simulink model "Papersimcurrentsource3"  (R2025a)
settings: Solver=ode23tb  StartTime=0.0  StopTime=0.3  MaxStep=5e-5  RelTol=1e-3
undefined symbols (not defined in the file): D11, Delta, I_PV_R_ML
libraries: spsRMSLib x20, spsCurrentMeasurementLib x5, spsParallelRLCLoadLib x4, spsACCurrentSourceLib x3, spsBreakerLib x3, spsPower3phInstantaneousLib x3, spsThreePhaseVIMeasurementLib x3, spsSequenceAnalyzerLib x2, simulink x1, spsMeanLib x1, spsPowerPhasorLib x1, eePowerMeasurement x1
settings Model: NumberOfSteps=2  Creator=ADMIN  LastModifiedBy=Ayush

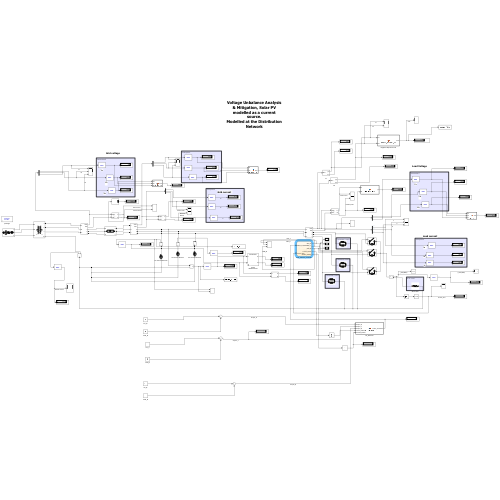
[thumbnail: Simulink's stored preview of the top-level diagram]
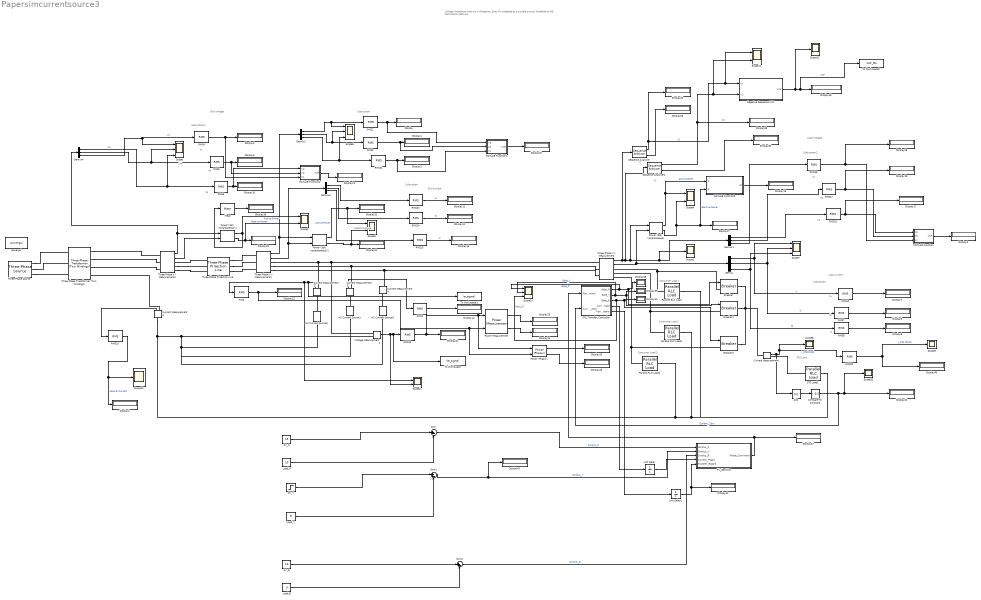
== system Papersimcurrentsource3 ==
  note: Gate_B
  note: Consumer Load 3
  note: Consumer Load 2
  note: STS Load
  note: Consumer Load 1
  note: Reactive Power
  note: V1
  note: Subsystem1
  note: Subsystem2
  note: Voltage Unbalance Analysis & Mitigation, Solar PV modelled as a current source.
      | Modelled at the Distribution Network
  note: Subsystem
  note: Subsystem
  note: Subsystem
  note: Ia
  note: Ib
  note: Ic
  note: Grid voltage
  note: Load current
  note: Load Voltage
  note: Vc
  note: Vb
  note: Va
  note: Vc
  note: Vb
  note: Va
  note: Grid current
  note: V2
  AC Current Source1 : spsACCurrentSourceLib/AC Current Source  Amplitude=20.86  Phase=-150  Frequency=50  SampleTime=0  Measurements=None
      settings: LibrarySourceBlock=sps_lib/Sources/AC Current Source
  AC Current Source2 : spsACCurrentSourceLib/AC Current Source  Amplitude=I_PV_R_ML  Phase=-30  Frequency=50  SampleTime=0  Measurements=None
      settings: LibrarySourceBlock=sps_lib/Sources/AC Current Source
  AC Current Source3 : spsACCurrentSourceLib/AC Current Source  Amplitude=40.86  Phase=90  Frequency=50  SampleTime=0  Measurements=None
      settings: LibrarySourceBlock=sps_lib/Sources/AC Current Source
  Abs : Abs  SaturateOnIntegerOverflow=off
  Breaker : spsBreakerLib/Breaker  InitialState=0  SwitchingTimes="[1/60  5/60]"  External=on  BreakerResistance=0.01  SnubberResistance=1e6  SnubberCapacitance=inf  Measurements=None  MoreParameters=on  NoBreakLoop=off
  Breaker1 : spsBreakerLib/Breaker  InitialState=0  SwitchingTimes="[1/60  5/60]"  External=on  BreakerResistance=0.01  SnubberResistance=1e6  SnubberCapacitance=inf  Measurements=None  MoreParameters=on  NoBreakLoop=off
  Breaker2 : spsBreakerLib/Breaker  InitialState=0  SwitchingTimes="[1/60  5/60]"  External=on  BreakerResistance=0.01  SnubberResistance=1e6  SnubberCapacitance=inf  Measurements=None  MoreParameters=on  NoBreakLoop=off
  Compare To Constant : simulink/Logic and Bit Operations/Compare To Constant  relop=<  const=0.5  OutDataTypeStr=boolean
  Current Measurement{,1..4} (5 alike) : spsCurrentMeasurementLib/Current Measurement  PhasorSimulation=off  OutputType=Complex  PSBequivalent=0
  Demux{,1..4} (5 alike) : Demux  Outputs=3
  Display{,1..27,29..40,42..46} (45 alike) : Display
  Load_B : Constant  Value=3
  Load_R : Constant  Value=10
  Load_Y : Constant  Value=5
  MATLAB Function : MATLAB Function  TreatAsAtomicUnit=on
  MATLAB Function1 : MATLAB Function  TreatAsAtomicUnit=on
  MATLAB Function2 : MATLAB Function  TreatAsAtomicUnit=on
  MATLAB Function3 : MATLAB Function  TreatAsAtomicUnit=on
  Mean : spsMeanLib/Mean  Freq=50  Vinit=0  Ts=0
  Negative-Sequence VUF : MATLAB Function  TreatAsAtomicUnit=on
  PV_B : Constant  Value=10
  PV_Decision : MATLAB Function  TreatAsAtomicUnit=on
  PV_R : Constant  Value=15
  PV_Y : Step  Time=0.1  After=10  SampleTime=0
  Parallel RLC Load : spsParallelRLCLoadLib/Parallel RLC Load  LConnTagsString=a  RConnTagsString=__new0  NominalVoltage=239.6  NominalFrequency=50  ActivePower=P_R_ML  InductivePower=0.0315e3  CapacitivePower=0  Setx0=off  InitialVoltage=0  SetiL0=off  InitialCurrent=0  Measurements=None  LoadType=constant PQ
      settings: AttributesFormatString=\n  LibrarySourceBlock=sps_lib/Passives/Parallel RLC Load
  Parallel RLC Load1 : spsParallelRLCLoadLib/Parallel RLC Load  LConnTagsString=a  RConnTagsString=__new0  NominalVoltage=239.6  NominalFrequency=50  ActivePower=P_Y_ML  InductivePower=0.1700e3  CapacitivePower=0  Setx0=off  InitialVoltage=0  SetiL0=off  InitialCurrent=0  Measurements=None  LoadType=constant PQ
      settings: AttributesFormatString=\n  LibrarySourceBlock=sps_lib/Passives/Parallel RLC Load
  Parallel RLC Load2 : spsParallelRLCLoadLib/Parallel RLC Load  LConnTagsString=a  RConnTagsString=__new0  NominalVoltage=239.6  NominalFrequency=50  ActivePower=P_B_ML  InductivePower=0.0416e3  CapacitivePower=0  Setx0=off  InitialVoltage=0  SetiL0=off  InitialCurrent=0  Measurements=None  LoadType=constant PQ
      settings: AttributesFormatString=\n  LibrarySourceBlock=sps_lib/Passives/Parallel RLC Load
  "Power (3ph, Instantaneous)" : spsPower3phInstantaneousLib/Power (3ph, Instantaneous)
  "Power (3ph, Instantaneous)1" : spsPower3phInstantaneousLib/Power (3ph, Instantaneous)
  "Power (3ph, Instantaneous)2" : spsPower3phInstantaneousLib/Power (3ph, Instantaneous)
  Power (Phasor) : spsPowerPhasorLib/Power (Phasor)
      settings: LibrarySourceBlock=|
      | sps_lib/Sensors and Measurements/Power
      | (Phasor)
  Power Measurement : eePowerMeasurement/Power Measurement  LabelModeActiveChoice=Continuous  F=50  K=[0 1 2 3]  Ts=0
  RMS{,1..3,10..11} (6 alike) : spsRMSLib/RMS  TrueRMS=on  Freq=50  RMSInit=120  Ts=0
  RMS{4..8,12..20} (14 alike) : spsRMSLib/RMS  TrueRMS=on  Freq=50  RMSInit=0  Ts=0
  STS Load1 : spsParallelRLCLoadLib/Parallel RLC Load  LConnTagsString=a  RConnTagsString=__new0  NominalVoltage=239.6  NominalFrequency=50  ActivePower=2e3  InductivePower=0  CapacitivePower=0  Setx0=off  InitialVoltage=0  SetiL0=off  InitialCurrent=0  Measurements=None  LoadType=constant PQ
      settings: AttributesFormatString=\n  LibrarySourceBlock=sps_lib/Passives/Parallel RLC Load
  STS_Transfer_Controller : Stateflow chart  TreatAsAtomicUnit=on
  Scope{,6..7,14} (4 alike) : Scope  NumInputPorts=3
      Scope settings: ActiveDisplayYMinimum=-425.43606031355353  ActiveDisplayYMaximum=425.43606031174352  DataLoggingVariableName=ScopeData3
      Scope14 settings: ActiveDisplayYMinimum=-0.16380790454043723  ActiveDisplayYMaximum=1.2059962338446713  DataLoggingVariableName=ScopeData14
      Scope6 settings: ActiveDisplayYMinimum=-20239.45233714371  ActiveDisplayYMaximum=45014.061236636866  DataLoggingVariableName=ScopeData6
      Scope7 settings: ActiveDisplayYMinimum=-71.559323570240508  ActiveDisplayYMaximum=80.121420785027254  DataLoggingVariableName=ScopeData7
  Scope{1,8..10,12..13} (6 alike) : Scope
      Scope1 settings: ActiveDisplayYMinimum=-426.70454804038366  ActiveDisplayYMaximum=427.02119643407605
      Scope10 settings: ActiveDisplayYMinimum=-0.038971823091303648  ActiveDisplayYMaximum=1.0948150249812589  DataLoggingVariableName=ScopeData10
      Scope12 settings: ActiveDisplayYMinimum=-1  ActiveDisplayYMaximum=1  DataLoggingVariableName=ScopeData12
      Scope13 settings: ActiveDisplayYMinimum=-3.2938329097835997  ActiveDisplayYMaximum=20.839767093612007  DataLoggingVariableName=ScopeData13
      Scope8 settings: ActiveDisplayYMinimum=-15.212573689341452  ActiveDisplayYMaximum=15.799802923178035  DataLoggingVariableName=ScopeData8
      Scope9 settings: ActiveDisplayYMinimum=0.40151551924009254  ActiveDisplayYMaximum=8.5834184270286613  DataLoggingVariableName=ScopeData9
  Scope{2..5,11} (5 alike) : Scope  NumInputPorts=2
      Scope11 settings: ActiveDisplayYMinimum=-1  ActiveDisplayYMaximum=1  DataLoggingVariableName=ScopeData11
      Scope2 settings: ActiveDisplayYMinimum=-389.69550713008283  ActiveDisplayYMaximum=420.87685595853827
      Scope3 settings: ActiveDisplayYMinimum=-14867.941772669114  ActiveDisplayYMaximum=35550.630177259292  DataLoggingVariableName=ScopeData2
      Scope4 settings: ActiveDisplayYMinimum=-211.09061912375623  ActiveDisplayYMaximum=673.0400671342187  DataLoggingVariableName=ScopeData4
      Scope5 settings: ActiveDisplayYMinimum=-32711.501465572641  ActiveDisplayYMaximum=66501.609586384555  DataLoggingVariableName=ScopeData5
  Sequence Analyzer : spsSequenceAnalyzerLib/Sequence Analyzer  Freq=50  n=1  seq=Positive  InInit=[1, 0]  Ts=0
      settings: LibrarySourceBlock=sps_lib/Sensors and Measurements/Sequence Analyzer
  Sequence Analyzer1 : spsSequenceAnalyzerLib/Sequence Analyzer  Freq=50  n=1  seq=Negative  InInit=[1, 0]  Ts=0
      settings: LibrarySourceBlock=sps_lib/Sensors and Measurements/Sequence Analyzer
  Sum : Sum  Inputs=|+-
  Sum1 : Sum  Inputs=|+-
  Sum2 : Sum  Inputs=|+-
  Three-Phase PI Section Line : spsThreePhasePISectionLineLib/Three-Phase PI Section Line  LConnTagsString=a|b|c  RConnTagsString=A|B|C  Length=1.5  Frequency=50  Resistances=[ 0.14 0.40]  Inductances=[ 1.0e-3 3.5e-3]  Capacitances=[11e-9 6e-9]
  Three-Phase Transformer (Two Windings) : spsThreePhaseTransformerTwoWindingsLib/Three-Phase Transformer (Two Windings)  Winding1Connection=Delta (D11)  Winding2Connection=Yn  CoreType=Three single-phase transformers  SetSaturation=off  Hysteresis=off  DataFile='hysteresis'  SetInitialFlux=off  Measurements=None  UNITS=pu  NominalPower=[ 630e3 , 50 ]  Winding1=[ 11e3 , 0.005 , 0.04 ]  Winding2=[ 415 , 0.005 , 0.04 ]  Rm=500  Lm=500  L0=0.5  Saturation=[ 0,0 ; 0.0024,1.2 ; 1.0,1.52 ]  InitialFluxes=[ 0.8 , -0.8 , 0.7 ]  BreakLoop=off  DiscreteSolver=Trapezoidal iterative  DataType=off  TransfoNumber=1
  Three-Phase V-I Measurement : spsThreePhaseVIMeasurementLib/Three-Phase V-I Measurement  VoltageMeasurement=phase-to-ground  SetLabelV=off  LabelV=Vabc  Vpu=off  VpuLL=off  CurrentMeasurement=yes  SetLabelI=off  LabelI=Iabc  Ipu=off  Pbase=100e6  Vbase=500e3  OutputType=Complex  PhasorSimulation=off  PSBequivalent=0
  Three-Phase V-I Measurement1 : spsThreePhaseVIMeasurementLib/Three-Phase V-I Measurement  VoltageMeasurement=phase-to-ground  SetLabelV=off  LabelV=Vabc  Vpu=off  VpuLL=off  CurrentMeasurement=yes  SetLabelI=off  LabelI=Iabc  Ipu=off  Pbase=100e6  Vbase=500e3  OutputType=Complex  PhasorSimulation=off  PSBequivalent=0
  Three-Phase V-I Measurement2 : spsThreePhaseVIMeasurementLib/Three-Phase V-I Measurement  VoltageMeasurement=phase-to-ground  SetLabelV=off  LabelV=Vabc  Vpu=off  VpuLL=off  CurrentMeasurement=yes  SetLabelI=off  LabelI=Iabc  Ipu=off  Pbase=100e6  Vbase=500e3  OutputType=Complex  PhasorSimulation=off  PSBequivalent=0
  Three-Phase Source : spsThreePhaseSourceLib/Three-Phase Source  InternalConnection=Yg  VoltagePhases=off  Voltage=11000  PhaseAngle=0  Voltage_phases=[25e3 25e3 25e3]/sqrt(3)  PhaseAngles_phases=[0 -120 +120]  Frequency=50  NonIdealSource=on  SpecifyImpedance=on  Resistance=0.01  Inductance=0.1  ShortCircuitLevel=10e6  BaseVoltage=11e3  XRratio=7  BusType=swing  Pref=10e3  Qref=0  Prefabc=[10e3, 10e3, 10e3]  Qrefabc=[0, 0, 0]  Qmin=-inf  Qmax=inf
  To Workspace : ToWorkspace  VariableName=Va_signal  SaveFormat=Structure With Time  SampleTime=-1
  To Workspace1 : ToWorkspace  VariableName=Ia_signal  SaveFormat=Structure With Time  SampleTime=-1
  To Workspace2 : ToWorkspace  VariableName=VUF_ML  SaveFormat=Timeseries  SampleTime=-1
  Unit Delay : UnitDelay  InitialCondition=1  SampleTime=-1  HasFrameUpgradeWarning=on
  Unit Delay1 : UnitDelay  SampleTime=-1  HasFrameUpgradeWarning=on
  Voltage Measurement2 : spsVoltageMeasurementLib/Voltage Measurement  PhasorSimulation=off  OutputType=Complex  PSBequivalent=0
  powergui : spspowerguiLib/powergui  Priority=1  SimulationMode=Discrete  SampleTime=5e-6  frequency=50  Iterations=50  frequencyindice=50  Pbase=100e6  ErrMax=1e-4  UnitsV=kV  UnitsW=MW  buscounter=0  FunctionMessages=off  echomessages=off  EnableUseOfTLC=off  CurrentSourceSwitches=off  DisableSnubberDevices=off  DisableRonSwitches=off  DisableVfSwitches=off  DisplayEquations=off  AutomaticDiscreteSolvers=off  SolverType=Tustin/Backward Euler (TBE)  Interpol=off  ExternalGateDelay=off  methode=off  Ts=100  x0status=blocks  SPID=on  SwTol=0  HookPort=off  NonlinearTolerance=1e-4  nMaxIteration=100  ContinueOnMaxIteration=off  RestoreLinks=warning  ResistiveCurrentMeasurement=off  Frange=[0:2:500]  Ylog=off  Xlog=on  ShowGrid=off  save=off  variable=ZData  structure=0  ZoomFFT=off  StartTime=0.0  cycles=1  DisplayStyle=1  fundamental=60  FreqAxis=off  MaxFrequency=1000  frequencyindicesteady=1  RmsSteady=1  display=off
  wires:
  Three-Phase V-I Measurement/1 -> Sequence Analyzer/1, Sequence Analyzer1/1, "Power (3ph, Instantaneous)"/1, Scope1/1, Demux1/1
  Three-Phase V-I Measurement/2 -> "Power (3ph, Instantaneous)"/2, Demux/1
  MATLAB Function/1(VUF) -> Display3/1
  Demux/3 -> RMS8/1, Scope7/3  "Ib"
  Demux/1 -> RMS12/1, Scope7/1  "Ir"
  Demux/2 -> RMS7/1, Scope7/2  "Iy"
  RMS7/1 -> Display8/1
  RMS8/1 -> Display6/1
  RMS12/1 -> Display7/1
  RMS/1 -> Power (Phasor)/2, Power Measurement/2, Display13/1
  Three-Phase V-I Measurement1/1 -> "Power (3ph, Instantaneous)2"/1, Demux2/1
  Three-Phase V-I Measurement1/2 -> "Power (3ph, Instantaneous)2"/2, Demux3/1
  Demux2/3 -> Scope6/3, RMS11/1
  Demux2/2 -> Scope6/2, RMS3/1
  RMS2/1 -> MATLAB Function1/1(Va), Display/1
  RMS3/1 -> MATLAB Function1/2(Vb), Display1/1
  Demux2/1 -> Scope6/1, RMS2/1
  RMS11/1 -> MATLAB Function1/3(Vc), Display2/1
  Demux3/3 -> RMS15/1
  RMS15/1 -> Display16/1  "Ic"
  Demux3/1 -> RMS13/1
  RMS14/1 -> Display12/1  "Ib"
  RMS13/1 -> Display11/1  "Ia"
  Demux3/2 -> RMS14/1
  Current Measurement2/1 -> RMS/1, Scope2/1, To Workspace1/1
  RMS1/1 -> Display14/1
  Current Measurement3/1 -> RMS1/1
  Demux4/2 -> Scope/2, RMS5/1  "Vb"
  Demux4/3 -> Scope/1, RMS4/1  "Vc"
  RMS4/1 -> MATLAB Function2/3(Vc), Display5/1
  Demux4/1 -> Scope/3, RMS6/1  "Va"
  RMS5/1 -> MATLAB Function2/2(Vb), Display9/1
  RMS6/1 -> MATLAB Function2/1(Va), Display10/1
  Three-Phase V-I Measurement2/1 -> "Power (3ph, Instantaneous)1"/1, Demux4/1
  Demux1/2 -> RMS17/1
  Demux1/3 -> RMS16/1
  Demux1/1 -> RMS18/1
  RMS10/1 -> Scope13/1, Display4/1  "Neutral Current"
  Current Measurement1/1 -> RMS10/1
  MATLAB Function1/1(VUF) -> Display20/1
  MATLAB Function2/1(VUF) -> Display21/1
  RMS19/1 -> Power (Phasor)/1, Power Measurement/1, Display22/1
  Voltage Measurement2/1 -> Scope2/2, To Workspace/1, RMS19/1
  Power Measurement/2 -> Display24/1
  Power (Phasor)/1 -> Display25/1
  Power (Phasor)/2 -> Display26/1
  "Power (3ph, Instantaneous)"/1 -> MATLAB Function3/1(P), Scope4/1  "active power"
  "Power (3ph, Instantaneous)"/2 -> Scope4/2, MATLAB Function3/2(Q), Display27/1  "reactive power"
  "Power (3ph, Instantaneous)1"/2 -> Scope3/2, Display29/1  "Passive Power"
  "Power (3ph, Instantaneous)1"/1 -> Scope3/1, Mean/1  "Active Power"
  Three-Phase V-I Measurement2/2 -> "Power (3ph, Instantaneous)1"/2
  "Power (3ph, Instantaneous)2"/2 -> Scope5/2, Display31/1
  "Power (3ph, Instantaneous)2"/1 -> Scope5/1, Display32/1  "Active Power"
  Sequence Analyzer1/2 -> Display35/1
  Mean/1 -> Display30/1
  Power Measurement/1 -> Display23/1
  RMS18/1 -> MATLAB Function/1(Va), Display17/1
  RMS17/1 -> MATLAB Function/2(Vb), Display19/1
  RMS16/1 -> MATLAB Function/3(Vc), Display18/1
  STS_Transfer_Controller/1(Gate_R) -> Scope14/1, Display38/1, Breaker/1  "Gate_R"
  STS_Transfer_Controller/2(Gate_Y) -> Scope14/2, Display39/1, Breaker1/1  "Gate_Y"
  STS_Transfer_Controller/3(Gate_B) -> Scope14/3, Display40/1, Breaker2/1
  Sum/1 -> PV_Decision/1(Surplus_R)  "Surplus_R"
  Sum1/1 -> Display43/1, PV_Decision/2(Surplus_Y)  "Surplus_Y"
  Load_R/1 -> Sum/2
  PV_R/1 -> Sum/1
  PV_Y/1 -> Sum1/1
  Load_Y/1 -> Sum1/2
  PV_B/1 -> Sum2/1
  Load_B/1 -> Sum2/2
  Sum2/1 -> PV_Decision/3(Surplus_B)  "Surplus_B"
  STS_Transfer_Controller/4(Current_Phase) -> Unit Delay/1
  Unit Delay/1 -> PV_Decision/4(Current_Phase)
  Unit Delay1/1 -> Display42/1, PV_Decision/5(Transfer_Enable)
  STS_Transfer_Controller/5(Transfer_Enable) -> Unit Delay1/1
  Abs/1 -> Compare To Constant/1
  Current Measurement/1 -> Abs/1, RMS20/1, Scope8/1  "I_STS(RMS)"
  RMS20/1 -> Scope9/1, Display44/1  "I_STS (RMS)"
  Compare To Constant/1 -> Scope10/1, Display45/1, STS_Transfer_Controller/2(Current_Zero)  "Current_Zero"
  Negative-Sequence VUF/1(VUF) -> Scope12/1, To Workspace2/1, Display46/1  "VUF"
  Sequence Analyzer/2 -> Display36/1
  Sequence Analyzer1/1 -> Scope11/2, Negative-Sequence VUF/2(V2), Display33/1  "V2"
  Sequence Analyzer/1 -> Scope11/1, Negative-Sequence VUF/1(V1), Display34/1  "V1"
  MATLAB Function3/1(pf) -> Display15/1
  PV_Decision/1(Phase_Command) -> Display37/1, STS_Transfer_Controller/1(Phase_Command)
  connections:
  Three-Phase V-I Measurement1/RConn1 -- Current Measurement2/RConn1 -- Voltage Measurement2/LConn1 -- Three-Phase V-I Measurement/LConn1
  Three-Phase V-I Measurement1/RConn2 -- Current Measurement3/RConn1 -- Three-Phase V-I Measurement/LConn2
  Three-Phase V-I Measurement1/RConn3 -- Current Measurement4/RConn1 -- Three-Phase V-I Measurement/LConn3
  AC Current Source2/RConn1 -- Current Measurement2/LConn1
  AC Current Source1/RConn1 -- Current Measurement3/LConn1
  AC Current Source3/RConn1 -- Current Measurement4/LConn1
  Three-Phase Transformer (Two Windings)/RConn1 -- Three-Phase V-I Measurement2/LConn1
  Three-Phase Transformer (Two Windings)/RConn2 -- Three-Phase V-I Measurement2/LConn2
  Three-Phase Transformer (Two Windings)/RConn3 -- Three-Phase V-I Measurement2/LConn3
  Three-Phase Source/RConn2 -- Three-Phase Transformer (Two Windings)/LConn2
  Three-Phase Source/RConn3 -- Three-Phase Transformer (Two Windings)/LConn3
  Three-Phase Source/RConn1 -- Three-Phase Transformer (Two Windings)/LConn1
  Parallel RLC Load/LConn1 -- Breaker/LConn1 -- Three-Phase V-I Measurement/RConn1
  Parallel RLC Load2/LConn1 -- Three-Phase V-I Measurement/RConn3 -- Breaker2/LConn1
  Parallel RLC Load1/LConn1 -- Three-Phase V-I Measurement/RConn2 -- Breaker1/LConn1
  Breaker/RConn1 -- Breaker2/RConn1 -- Current Measurement/LConn1 -- Breaker1/RConn1
  Current Measurement/RConn1 -- STS Load1/LConn1
  Current Measurement1/RConn1 -- Three-Phase Transformer (Two Windings)/RConn4
  Parallel RLC Load1/RConn1 -- STS Load1/RConn1 -- Parallel RLC Load/RConn1 -- Parallel RLC Load2/RConn1 -- Current Measurement1/LConn1 -- Voltage Measurement2/LConn2 -- AC Current Source3/LConn1 -- AC Current Source1/LConn1 -- AC Current Source2/LConn1
  Three-Phase V-I Measurement2/RConn1 -- Three-Phase PI Section Line/LConn1
  Three-Phase V-I Measurement2/RConn2 -- Three-Phase PI Section Line/LConn2
  Three-Phase V-I Measurement2/RConn3 -- Three-Phase PI Section Line/LConn3
  Three-Phase PI Section Line/RConn1 -- Three-Phase V-I Measurement1/LConn1
  Three-Phase PI Section Line/RConn2 -- Three-Phase V-I Measurement1/LConn2
  Three-Phase PI Section Line/RConn3 -- Three-Phase V-I Measurement1/LConn3

== matlab function Papersimcurrentsource3/Negative-Sequence VUF ==
  data: V1 input; VUF output; V2 input
function VUF = compute_sequence_vuf(V1, V2)

VUF = 100 * abs(V2) / max(abs(V1), 1e-6);

end

== matlab function Papersimcurrentsource3/MATLAB Function3 ==
  data: P input; pf output; Q input
function pf = calcPowerFactor(P, Q)
    % P: Active Power (W or kW)
    % Q: Reactive Power (VAR or kVAR)
    % pf: Power Factor (0 to 1)

    % Apparent Power
    S = sqrt(P^2 + Q^2);

    % Prevent division by zero when both P and Q are zero
    if S == 0
        pf = 1.0; 
    else
        pf = abs(P) / S;
    end
end

== matlab function Papersimcurrentsource3/MATLAB Function1 ==
  data: Va input; VUF output; Vb input; Vc input
function VUF = compute_vuf(Va, Vb, Vc)
Vavg = (abs(Va) + abs(Vb) + abs(Vc)) / 3;
VUF = max([abs(abs(Va)-Vavg), ...
           abs(abs(Vb)-Vavg), ...
           abs(abs(Vc)-Vavg)]) / Vavg * 100;
end

== matlab function Papersimcurrentsource3/MATLAB Function ==
  data: Va input; VUF output; Vb input; Vc input
function VUF = compute_vuf(Va, Vb, Vc)
Vavg = (abs(Va) + abs(Vb) + abs(Vc)) / 3;
VUF = max([abs(abs(Va)-Vavg), ...
           abs(abs(Vb)-Vavg), ...
           abs(abs(Vc)-Vavg)]) / Vavg * 100;
end

== matlab function Papersimcurrentsource3/MATLAB Function2 ==
  data: Va input; VUF output; Vb input; Vc input
function VUF = compute_vuf(Va, Vb, Vc)
Vavg = (abs(Va) + abs(Vb) + abs(Vc)) / 3;
VUF = max([abs(abs(Va)-Vavg), ...
           abs(abs(Vb)-Vavg), ...
           abs(abs(Vc)-Vavg)]) / Vavg * 100;
end

== stateflow chart Papersimcurrentsource3/STS_Transfer_Controller ==
  state B_ACTIVE
    entry:
    Gate_R = 0;
    Gate_Y = 0;
    Gate_B = 1;
    Current_Phase = 3;
    Transfer_Enable = 0;
    during:
    if after(50,msec)
    Transfer_Enable = 1;
    end
  state Y_ACTIVE
    entry:
    Gate_R = 0;
    Gate_Y = 1;
    Gate_B = 0;
    Current_Phase = 2;
    Transfer_Enable = 0;
    during:
    if after(50,msec)
    Transfer_Enable = 1;
    end
  state R_ACTIVE
    entry:
    Gate_R = 1;
    Gate_Y = 0;
    Gate_B = 0;
    Current_Phase = 1;
    Transfer_Enable = 0;
    during:
    if after(50,msec)
    Transfer_Enable = 1;
    end
  state WAIT_ZERO
    entry:
    Gate_R = 0;
    Gate_Y = 0;
    Gate_B = 0;
    Transfer_Enable = 0;
  state DEAD_TIME
    entry:
    Gate_R = 0;
    Gate_Y = 0;
    Gate_B = 0;
    Transfer_Enable = 0;
  (default) -> Y_ACTIVE
  B_ACTIVE -> WAIT_ZERO : [Phase_Command ~= 3]{Target_Phase = Phase_Command;}
  DEAD_TIME -> B_ACTIVE [order 1] : [after(10,msec) && Target_Phase == 3]
  Y_ACTIVE -> WAIT_ZERO : [Phase_Command ~= 2]{Target_Phase = Phase_Command;}
  DEAD_TIME -> Y_ACTIVE [order 2] : [after(10,msec) && Target_Phase == 2]
  DEAD_TIME -> R_ACTIVE [order 3] : [after(10,msec) && Target_Phase == 1]
  R_ACTIVE -> WAIT_ZERO : [Phase_Command ~= 1]{Target_Phase = Phase_Command;}
  WAIT_ZERO -> DEAD_TIME : [Current_Zero == 1]
  data: Gate_R output =0; Gate_Y output =0; Phase_Command input; Gate_B output =0; Current_Phase output =1; Transfer_Enable output =0; Current_Zero input; Target_Phase local =1

== matlab function Papersimcurrentsource3/PV_Decision ==
  data: Surplus_R input; Phase_Command output; Surplus_Y input; Surplus_B input; Current_Phase input; Transfer_Enable input
function Phase_Command = PV_Decision( ...
    Surplus_R, Surplus_Y, Surplus_B, ...
    Current_Phase, Transfer_Enable)

PV_Threshold = 2;       % kW
Transfer_Margin = 1;    % kW

% Dwell time not completed:
% do not permit another phase transfer

if Transfer_Enable == 0
    Phase_Command = Current_Phase;
    return;
end

Max_Surplus = max([Surplus_R, Surplus_Y, Surplus_B]);

% No excessive PV
if Max_Surplus <= PV_Threshold
    Phase_Command = Current_Phase;
    return;
end

% Present phase surplus
if Current_Phase == 1
    Current_Surplus = Surplus_R;
elseif Current_Phase == 2
    Current_Surplus = Surplus_Y;
else
    Current_Surplus = Surplus_B;
end

% Hysteresis / transfer margin
if Max_Surplus <= (Current_Surplus + Transfer_Margin)
    Phase_Command = Current_Phase;
    return;
end

% Select phase with maximum PV surplus
if Surplus_R == Max_Surplus
    Phase_Command = 1;
elseif Surplus_Y == Max_Surplus
    Phase_Command = 2;
else
    Phase_Command = 3;
end
